simulink model "MCU_Sensing"  (R2024a)
settings: Solver=FixedStepDiscrete  StartTime=0.0  StopTime=0.0001  FixedStep=1e-7  RelTol=1e-3
libraries: fl_lib x11, slpidlib x3, simulink x3, nesl_utility x3, spsPWMGeneratorDCDCLib x1, ee_lib x1
settings Model: Creator=g_lautur  LastModifiedBy=g_lautur

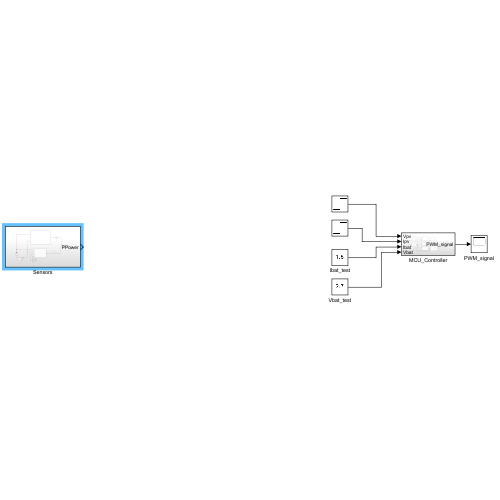
[thumbnail: Simulink's stored preview of the top-level diagram]
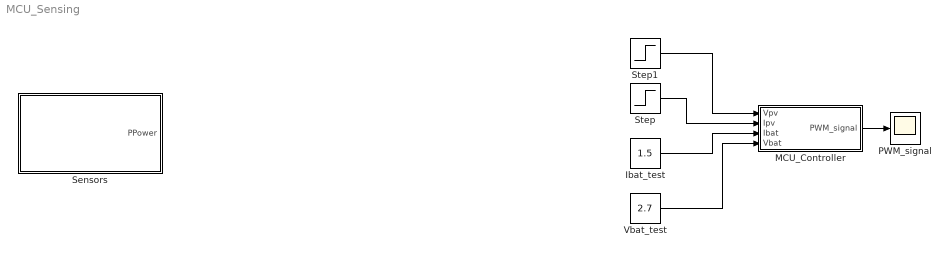
== system MCU_Sensing ==
  Ibat_test : Constant  Value=1.5
  MCU_Controller : Subsystem
  PWM_signal : Scope
  Sensors : Subsystem
  Step : Step  Time=2  Before=1.248  After=1.30  SampleTime=0
  Step1 : Step  Time=2  Before=2.0625  After=2.125  SampleTime=0
  Vbat_test : Constant  Value=2.7
  wires:
  Step1/1 -> MCU_Controller/1(Vpv)
  Step/1 -> MCU_Controller/2(Ipv)
  Vbat_test/1 -> MCU_Controller/4(Vbat)
  Ibat_test/1 -> MCU_Controller/3(Ibat)
  MCU_Controller/1(PWM_signal) -> PWM_signal/1

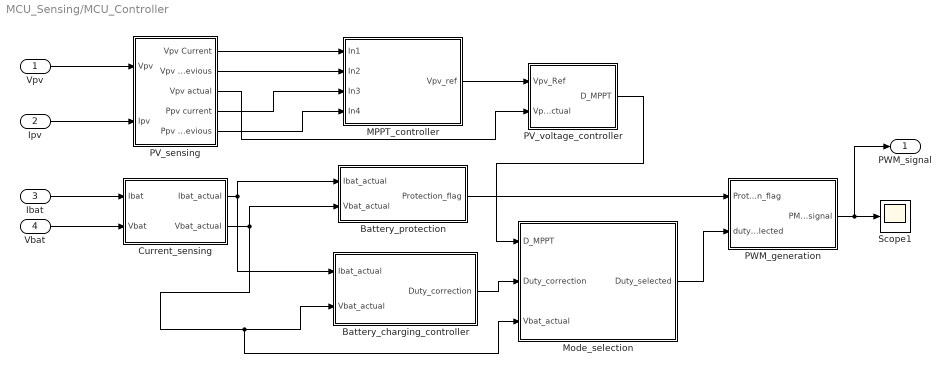
== system MCU_Sensing/MCU_Controller ==
  Vpv : Inport
  Ipv : Inport  Port=2
  Ibat : Inport  Port=3
  Vbat : Inport  Port=4
  Battery_charging_controller : Subsystem
  Battery_protection : Subsystem
  Current_sensing : Subsystem
  MPPT_controller : Subsystem
  Mode_selection : Subsystem
  PV_sensing : Subsystem
  PV_voltage_controller : Subsystem
  PWM_generation : Subsystem
  Scope1 : Scope
  PWM_signal : Outport
  wires:
  Vpv/1 -> PV_sensing/1(Vpv)
  Ipv/1 -> PV_sensing/2(Ipv)
  PV_sensing/1(Vpv Current) -> MPPT_controller/1(In1)
  PV_sensing/2(Vpv Previous) -> MPPT_controller/2(In2)
  PV_sensing/4(Ppv current) -> MPPT_controller/3(In3)
  PV_sensing/5(Ppv previous) -> MPPT_controller/4(In4)
  MPPT_controller/1(Vpv_ref) -> PV_voltage_controller/1(Vpv_Ref)
  PV_sensing/3(Vpv actual) -> PV_voltage_controller/2(Vpv_actual)
  Current_sensing/1(Ibat_actual) -> Battery_charging_controller/1(Ibat_actual), Battery_protection/1(Ibat_actual)
  Current_sensing/2(Vbat_actual) -> Battery_charging_controller/2(Vbat_actual), Mode_selection/3(Vbat_actual), Battery_protection/2(Vbat_actual)
  Ibat/1 -> Current_sensing/1(Ibat)
  Vbat/1 -> Current_sensing/2(Vbat)
  PV_voltage_controller/1(D_MPPT) -> Mode_selection/1(D_MPPT)
  Battery_charging_controller/1(Duty_correction) -> Mode_selection/2(Duty_correction)
  Battery_protection/1(Protection_flag) -> PWM_generation/1(Protection_flag)
  Mode_selection/1(Duty_selected) -> PWM_generation/2(duty_selected)
  PWM_generation/1(PMW_signal) -> PWM_signal/1, Scope1/1

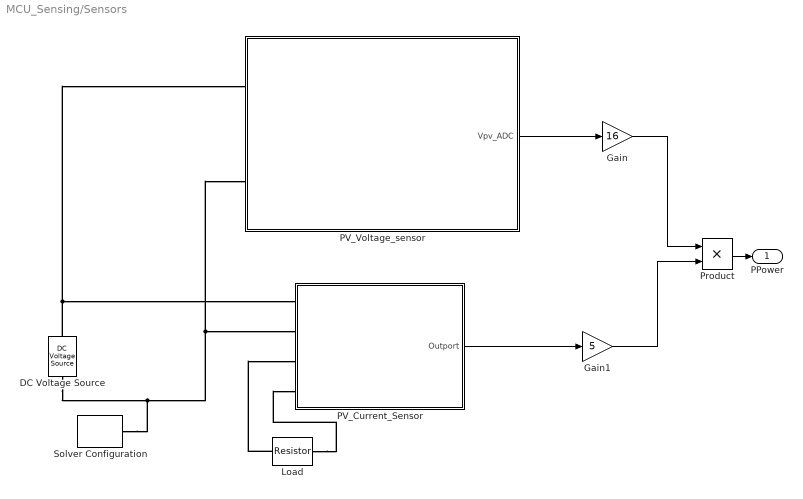
== system MCU_Sensing/Sensors ==
  DC Voltage Source : ee_lib/Additional Components/SPICE Sources/DC Voltage Source  DC=33 V
  Gain : Gain  Gain=16
  Gain1 : Gain  Gain=5
  Load : fl_lib/Electrical/Electrical Elements/Resistor  R=3.3 Ohm  i_specify=off  i_priority=None  i=0 A  i_nominal_specify=off  i_nominal_value=1  i_nominal_unit=A  v_specify=off  v_priority=None  v=0 V  v_nominal_specify=off  v_nominal_value=1  v_nominal_unit=V
  PV_Current_Sensor : Subsystem
  PV_Voltage_sensor : Subsystem
  Product : Product
  Solver Configuration : nesl_utility/Solver Configuration  PhysicalDomain=network_engine_domain  SubClassName=solver  LeftPortType=input  RightPortType=generic  Tones=[]  Harmonics=[]  SimulateNoise=off  Profile=off  UseLocalSampling=off  EnableSwitchedLinearOptims=on  FrequencyDomain=off  UseCCode=off  RelTol=0.001  AbsTol=0.001  MinStep=1e-09  ToWorkspace=off  RevertToSquareIcSolve=off  NumHomotopyIterations=100  PhasorMode=off  PhasorModeNumHarmonics=1  ConsistencySolver=NEWTON_XTOL_AFTER_FTOL  IndexReductionMethod=DerivativeReplacement  DoDC=off  ResidualTolerance=1e-09  ConsistencyTolSource=GLOBAL  ConsistencyAbsTol=0.001  ConsistencyRelTol=0.001  ConsistencyTolFactor=0.001  UseLocalSolver=off  LocalSolverChoice=NE_BACKWARD_EULER_ADVANCER  ResolveIndetEquations=on  FunctionEvalNumThread=1  LocalSolverSampleTime=0.001  DoFixedCost=off  MaxNonlinIter=3  MaxModeIter=2  ComputeImpulses=off  ImpulseIterations=2  LinearAlgebra=auto  LinearAlgebraNumThread=0  EquationFormulation=NE_TIME_EF  DelaysMemoryBudget=1024  AutomaticFiltering=on  FilteringTimeConstant=0.001  PartitionStorageMethod=AS_NEEDED  PartitionMemoryBudget=1024  PartitionMethod=ROBUST  MultibodyUseLocalSolver=off  MultibodyLocalSolverChoice=ODE1  MultibodyLocalSolverSampleTime=0.001
  PPower : Outport
  wires:
  PV_Current_Sensor/1(Outport) -> Gain1/1
  PV_Voltage_sensor/1(Vpv_ADC) -> Gain/1
  Gain1/1 -> Product/2
  Gain/1 -> Product/1
  Product/1 -> PPower/1
  connections:
  Load/RConn1 -- PV_Current_Sensor/LConn4
  DC Voltage Source/LConn1 -- PV_Current_Sensor/LConn1 -- PV_Voltage_sensor/LConn1
  Load/LConn1 -- PV_Current_Sensor/LConn3
  DC Voltage Source/RConn1 -- Solver Configuration/RConn1 -- PV_Current_Sensor/LConn2 -- PV_Voltage_sensor/LConn2

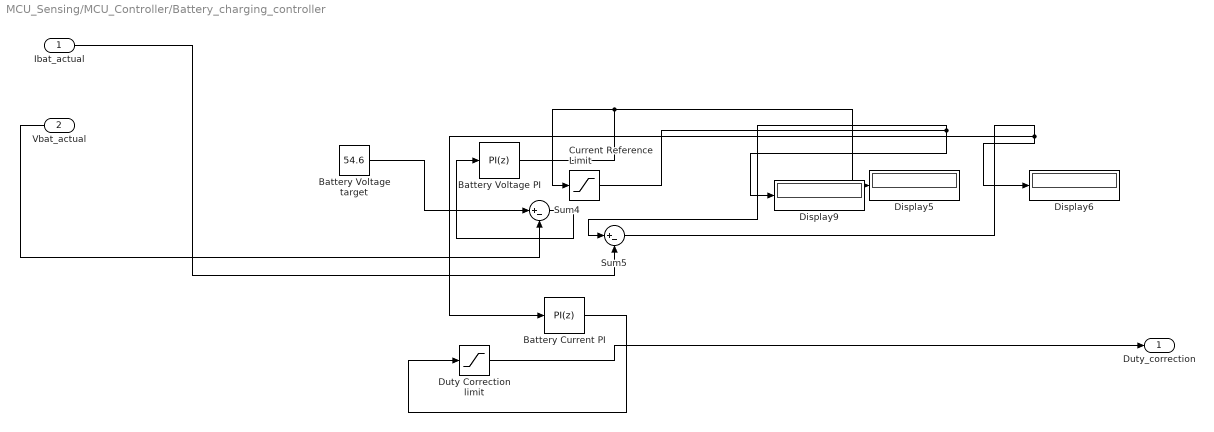
== system MCU_Sensing/MCU_Controller/Battery_charging_controller ==
  Ibat_actual : Inport
  Vbat_actual : Inport  Port=2
  "Battery Current PI " : slpidlib/PID Controller  Controller=PI  Form=Parallel  TimeDomain=Discrete-time  UseExternalTs=off  SampleTime=1e-5  IntegratorMethod=Forward Euler  FilterMethod=Forward Euler  ControllerParametersSource=internal  P=0.01  I=0.1  UseKiTs=off  D=0  UseExternalDerivativeSource=off  N=100  UseFilter=on  TunerSelectOption=Transfer Function Based (PID Tuner App)  InitialConditionSource=internal  InitialConditionForIntegrator=0  InitialConditionForFilter=0  DifferentiatorICPrevScaledInput=0  ExternalReset=none  TrackingMode=off  Kt=1  LimitOutput=off  SatLimitsSource=internal  UpperSaturationLimit=inf  LowerSaturationLimit=-inf  LinearizeAsGain=off  AntiWindupMode=none  Kb=1  LimitIntegrator=off  UpperIntegratorSaturationLimit=inf  LowerIntegratorSaturationLimit=-inf  POutMin=[]  POutMax=[]  IOutMin=[]  IOutMax=[]  DOutMin=[]  DOutMax=[]  NOutMin=[]  NOutMax=[]  SumOutMin=[]  SumOutMax=[]  SaturationOutMin=[]  SaturationOutMax=[]  PParamMin=[]  PParamMax=[]  IParamMin=[]  IParamMax=[]  DParamMin=[]  DParamMax=[]  NParamMin=[]  NParamMax=[]  KbParamMin=[]  KbParamMax=[]  KtParamMin=[]  KtParamMax=[]  KbOutMin=[]  KbOutMax=[]  KtOutMin=[]  KtOutMax=[]  IntegratorOutMin=[]  IntegratorOutMax=[]  FilterOutMin=[]  FilterOutMax=[]  SumI1OutMin=[]  SumI1OutMax=[]  SumI2OutMin=[]  SumI2OutMax=[]  SumI3OutMin=[]  SumI3OutMax=[]  SumI4OutMin=[]  SumI4OutMax=[]  SumDOutMin=[]  SumDOutMax=[]  DifferentiatorOutMin=[]  DifferentiatorOutMax=[]  FilterDiffOutCoefMin=[]  FilterDiffOutCoefMax=[]  ReciprocalOutMin=[]  ReciprocalOutMax=[]  SumDenOutMin=[]  SumDenOutMax=[]  SumNumOutMin=[]  SumNumOutMax=[]  DivideOutMin=[]  DivideOutMax=[]  UdiffTsProdOutMin=[]  UdiffTsProdOutMax=[]  NTsProdOutMin=[]  NTsProdOutMax=[]  UintegralTsProdOutMin=[]  UintegralTsProdOutMax=[]  UngainTsProdOutMin=[]  UngainTsProdOutMax=[]  ClampingZeroOutDataTypeStr=Inherit: Inherit via back propagation  ClampingZeroOutMin=[]  ClampingZeroOutMax=[]  FilterDenConstantOutDataTypeStr=Inherit: Inherit via back propagation  FilterDenConstantOutMin=[]  FilterDenConstantOutMax=[]  PCopyOutDataTypeStr=Inherit: Inherit via back propagation  PCopyOutMin=[]  PCopyOutMax=[]  NCopyOutDataTypeStr=Inherit: Inherit via back propagation  NCopyOutMin=[]  NCopyOutMax=[]  IntegratorContinuousStateAttributes=''  IntegratorStateMustResolveToSignalObject=off  IntegratorRTWStateStorageClass=Auto  FilterContinuousStateAttributes=''  FilterStateMustResolveToSignalObject=off  FilterRTWStateStorageClass=Auto  ParallelPVariant=InternalParameters  IdealPVariant=Disabled  IVariant=InternalParameters  DVariant=Disabled  IntegratorVariant=Discrete  SatVariant=Disabled  AWVariant=Passthrough  PCopyVariant=Disabled  TRVariant=Disabled  FdbkBlocksVariant=Forward  IdealPFdbkVariant=Disabled  SatFdbkVariant=Disabled  DerivativeFilterVariant=Disabled  NVariant=Disabled  NCopyVariant=Disabled_SignalSpec  FilterICVariant=Disabled  IntegratorICVariant=InternalICs  ExternalResetVariant=Disabled  TRSumVariant=Passthrough  SumFdbkVariant=Disabled  SumVariant=Sum_PI  TsampFilterVariant=InternalTs  TsampNgainVariant=Passthrough  TsampIntegralVariant=Disabled_SignalSpec  ExternalSaturationOutDataTypeStr=Inherit: Same as second input  DerivativeSourceVariant=Disabled
      settings: LibrarySourceBlock=simulink/Discrete/Discrete PID Controller
  Battery Voltage PI : slpidlib/PID Controller  Controller=PI  Form=Parallel  TimeDomain=Discrete-time  UseExternalTs=off  SampleTime=1e-5  IntegratorMethod=Forward Euler  FilterMethod=Forward Euler  ControllerParametersSource=internal  P=2  I=0.1  UseKiTs=off  D=0  UseExternalDerivativeSource=off  N=100  UseFilter=on  TunerSelectOption=Transfer Function Based (PID Tuner App)  InitialConditionSource=internal  InitialConditionForIntegrator=0  InitialConditionForFilter=0  DifferentiatorICPrevScaledInput=0  ExternalReset=none  TrackingMode=off  Kt=1  LimitOutput=off  SatLimitsSource=internal  UpperSaturationLimit=inf  LowerSaturationLimit=-inf  LinearizeAsGain=off  AntiWindupMode=none  Kb=1  LimitIntegrator=off  UpperIntegratorSaturationLimit=inf  LowerIntegratorSaturationLimit=-inf  POutMin=[]  POutMax=[]  IOutMin=[]  IOutMax=[]  DOutMin=[]  DOutMax=[]  NOutMin=[]  NOutMax=[]  SumOutMin=[]  SumOutMax=[]  SaturationOutMin=[]  SaturationOutMax=[]  PParamMin=[]  PParamMax=[]  IParamMin=[]  IParamMax=[]  DParamMin=[]  DParamMax=[]  NParamMin=[]  NParamMax=[]  KbParamMin=[]  KbParamMax=[]  KtParamMin=[]  KtParamMax=[]  KbOutMin=[]  KbOutMax=[]  KtOutMin=[]  KtOutMax=[]  IntegratorOutMin=[]  IntegratorOutMax=[]  FilterOutMin=[]  FilterOutMax=[]  SumI1OutMin=[]  SumI1OutMax=[]  SumI2OutMin=[]  SumI2OutMax=[]  SumI3OutMin=[]  SumI3OutMax=[]  SumI4OutMin=[]  SumI4OutMax=[]  SumDOutMin=[]  SumDOutMax=[]  DifferentiatorOutMin=[]  DifferentiatorOutMax=[]  FilterDiffOutCoefMin=[]  FilterDiffOutCoefMax=[]  ReciprocalOutMin=[]  ReciprocalOutMax=[]  SumDenOutMin=[]  SumDenOutMax=[]  SumNumOutMin=[]  SumNumOutMax=[]  DivideOutMin=[]  DivideOutMax=[]  UdiffTsProdOutMin=[]  UdiffTsProdOutMax=[]  NTsProdOutMin=[]  NTsProdOutMax=[]  UintegralTsProdOutMin=[]  UintegralTsProdOutMax=[]  UngainTsProdOutMin=[]  UngainTsProdOutMax=[]  ClampingZeroOutDataTypeStr=Inherit: Inherit via back propagation  ClampingZeroOutMin=[]  ClampingZeroOutMax=[]  FilterDenConstantOutDataTypeStr=Inherit: Inherit via back propagation  FilterDenConstantOutMin=[]  FilterDenConstantOutMax=[]  PCopyOutDataTypeStr=Inherit: Inherit via back propagation  PCopyOutMin=[]  PCopyOutMax=[]  NCopyOutDataTypeStr=Inherit: Inherit via back propagation  NCopyOutMin=[]  NCopyOutMax=[]  IntegratorContinuousStateAttributes=''  IntegratorStateMustResolveToSignalObject=off  IntegratorRTWStateStorageClass=Auto  FilterContinuousStateAttributes=''  FilterStateMustResolveToSignalObject=off  FilterRTWStateStorageClass=Auto  ParallelPVariant=InternalParameters  IdealPVariant=Disabled  IVariant=InternalParameters  DVariant=Disabled  IntegratorVariant=Discrete  SatVariant=Disabled  AWVariant=Passthrough  PCopyVariant=Disabled  TRVariant=Disabled  FdbkBlocksVariant=Forward  IdealPFdbkVariant=Disabled  SatFdbkVariant=Disabled  DerivativeFilterVariant=Disabled  NVariant=Disabled  NCopyVariant=Disabled_SignalSpec  FilterICVariant=Disabled  IntegratorICVariant=InternalICs  ExternalResetVariant=Disabled  TRSumVariant=Passthrough  SumFdbkVariant=Disabled  SumVariant=Sum_PI  TsampFilterVariant=InternalTs  TsampNgainVariant=Passthrough  TsampIntegralVariant=Disabled_SignalSpec  ExternalSaturationOutDataTypeStr=Inherit: Same as second input  DerivativeSourceVariant=Disabled
      settings: LibrarySourceBlock=simulink/Discrete/Discrete PID Controller
  Battery Voltage target : Constant  Value=54.6
  Current Reference Limit : Saturate  UpperLimit=8  LowerLimit=0
  Display5 : Display
  Display6 : Display
  Display9 : Display
  Duty Correction limit : Saturate  UpperLimit=0.8  LowerLimit=-0.8
  Sum4 : Sum  Inputs=|+-
  Sum5 : Sum  Inputs=|+-
  Duty_correction : Outport
  wires:
  Sum4/1 -> Battery Voltage PI/1
  Battery Voltage PI/1 -> Display5/1, Current Reference Limit/1
  Duty Correction limit/1 -> Duty_correction/1
  Battery Voltage target/1 -> Sum4/1
  Current Reference Limit/1 -> Sum5/1, Display9/1
  Sum5/1 -> "Battery Current PI "/1, Display6/1
  "Battery Current PI "/1 -> Duty Correction limit/1
  Ibat_actual/1 -> Sum5/2
  Vbat_actual/1 -> Sum4/2

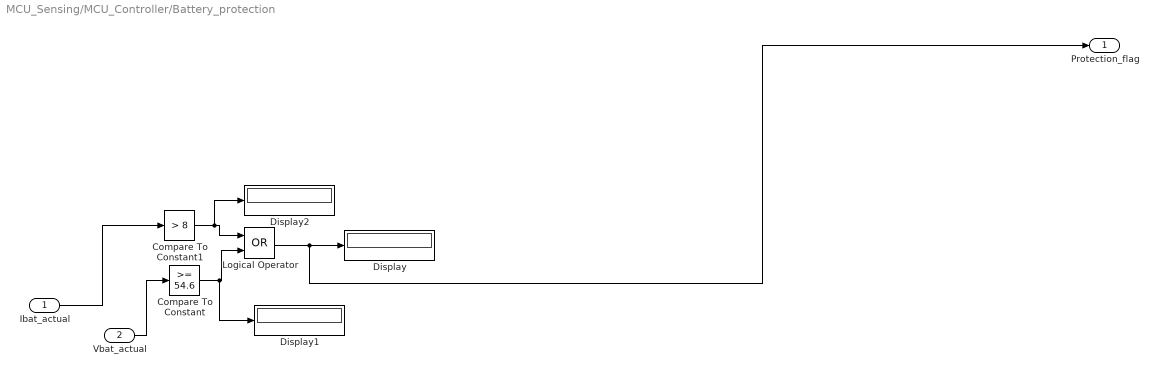
== system MCU_Sensing/MCU_Controller/Battery_protection ==
  Ibat_actual : Inport
  Vbat_actual : Inport  Port=2
  Compare To Constant : simulink/Logic and Bit Operations/Compare To Constant  relop=>=  const=54.6  OutDataTypeStr=boolean
  Compare To Constant1 : simulink/Logic and Bit Operations/Compare To Constant  relop=>  const=8  OutDataTypeStr=boolean  ZeroCross=off
  Display : Display
  Display1 : Display
  Display2 : Display
  Logical Operator : Logic  Operator=OR  AllPortsSameDT=off  OutDataTypeStr=boolean
  Protection_flag : Outport
  wires:
  Compare To Constant/1 -> Display1/1, Logical Operator/2
  Compare To Constant1/1 -> Display2/1, Logical Operator/1
  Logical Operator/1 -> Protection_flag/1, Display/1
  Vbat_actual/1 -> Compare To Constant/1
  Ibat_actual/1 -> Compare To Constant1/1

== system MCU_Sensing/MCU_Controller/Current_sensing ==
  Ibat : Inport
  Vbat : Inport  Port=2
  Gain2 : Gain  Gain=5
  Gain3 : Gain  Gain=20
  Ibat_actual : Outport
  Vbat_actual : Outport  Port=2
  wires:
  Gain3/1 -> Vbat_actual/1
  Vbat/1 -> Gain3/1
  Gain2/1 -> Ibat_actual/1
  Ibat/1 -> Gain2/1

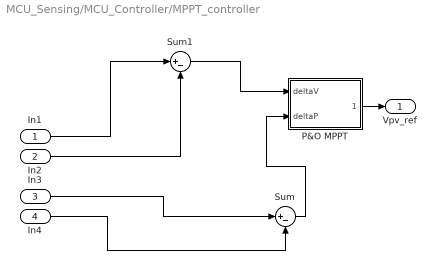
== system MCU_Sensing/MCU_Controller/MPPT_controller ==
  In1 : Inport
  In2 : Inport  Port=2
  In3 : Inport  Port=3
  In4 : Inport  Port=4
  P&O MPPT : MATLAB Function  TreatAsAtomicUnit=on
  Sum : Sum  Inputs=|+-
  Sum1 : Sum  Inputs=|+-
  Vpv_ref : Outport
  wires:
  Sum/1 -> P&O MPPT/2(deltaP)
  Sum1/1 -> P&O MPPT/1(deltaV)
  In4/1 -> Sum/2
  In1/1 -> Sum1/1
  P&O MPPT/1(Vpv_ref) -> Vpv_ref/1
  In3/1 -> Sum/1
  In2/1 -> Sum1/2

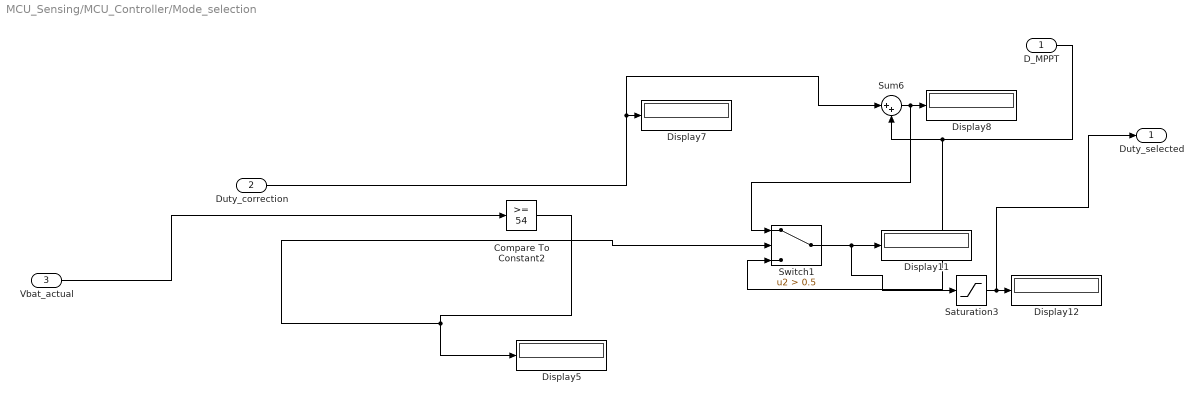
== system MCU_Sensing/MCU_Controller/Mode_selection ==
  D_MPPT : Inport
  Duty_correction : Inport  Port=2
  Vbat_actual : Inport  Port=3
  Compare To Constant2 : simulink/Logic and Bit Operations/Compare To Constant  relop=>=  const=54  OutDataTypeStr=boolean
  Display{5,7..8,11..12} (5 alike) : Display
  Saturation3 : Saturate  UpperLimit=0.8  LowerLimit=0
  Sum6 : Sum  Inputs=|++
  Switch1 : Switch  Criteria=u2 > Threshold  Threshold=0.5  SaturateOnIntegerOverflow=off  InputSameDT=off
  Duty_selected : Outport
  wires:
  D_MPPT/1 -> Switch1/3, Sum6/2
  Sum6/1 -> Switch1/1, Display8/1
  Vbat_actual/1 -> Compare To Constant2/1
  Duty_correction/1 -> Sum6/1, Display7/1
  Compare To Constant2/1 -> Display5/1, Switch1/2
  Switch1/1 -> Saturation3/1, Display11/1
  Saturation3/1 -> Duty_selected/1, Display12/1

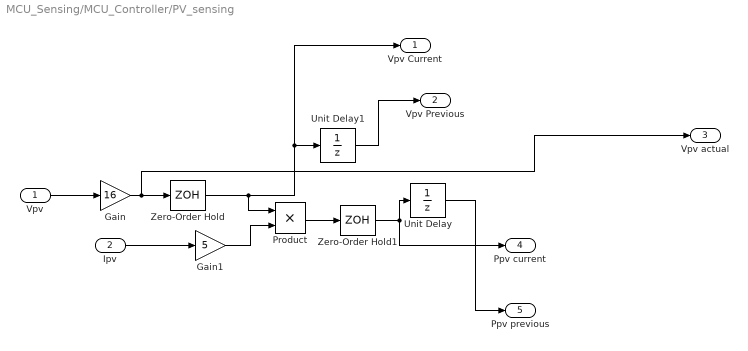
== system MCU_Sensing/MCU_Controller/PV_sensing ==
  Vpv : Inport
  Ipv : Inport  Port=2
  Gain : Gain  Gain=16
  Gain1 : Gain  Gain=5
  Product : Product
  Unit Delay : UnitDelay  InitialCondition=205.92  SampleTime=0.1  HasFrameUpgradeWarning=on
  Unit Delay1 : UnitDelay  InitialCondition=33  SampleTime=0.1  HasFrameUpgradeWarning=on
  Zero-Order Hold : ZeroOrderHold  SampleTime=0.1
  Zero-Order Hold1 : ZeroOrderHold  SampleTime=0.1
  Vpv Current : Outport
  Vpv Previous : Outport  Port=2
  Vpv actual : Outport  Port=3
  Ppv current : Outport  Port=4
  Ppv previous : Outport  Port=5
  wires:
  Product/1 -> Zero-Order Hold1/1
  Zero-Order Hold/1 -> Vpv Current/1, Unit Delay1/1, Product/1
  Unit Delay/1 -> Ppv previous/1
  Gain/1 -> Vpv actual/1, Zero-Order Hold/1
  Ipv/1 -> Gain1/1
  Gain1/1 -> Product/2
  Vpv/1 -> Gain/1
  Zero-Order Hold1/1 -> Ppv current/1, Unit Delay/1
  Unit Delay1/1 -> Vpv Previous/1

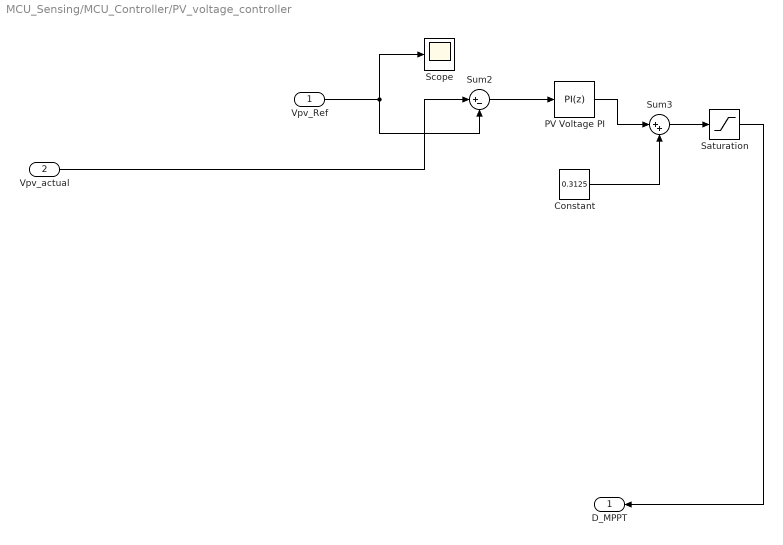
== system MCU_Sensing/MCU_Controller/PV_voltage_controller ==
  Vpv_Ref : Inport
  Vpv_actual : Inport  Port=2
  Constant : Constant  Value=0.3125
  PV Voltage PI : slpidlib/PID Controller  Controller=PI  Form=Parallel  TimeDomain=Discrete-time  UseExternalTs=off  SampleTime=0.1  IntegratorMethod=Forward Euler  FilterMethod=Forward Euler  ControllerParametersSource=internal  P=0.001  I=0.01  UseKiTs=off  D=0  UseExternalDerivativeSource=off  N=100  UseFilter=on  TunerSelectOption=Transfer Function Based (PID Tuner App)  InitialConditionSource=internal  InitialConditionForIntegrator=0  InitialConditionForFilter=0  DifferentiatorICPrevScaledInput=0  ExternalReset=none  TrackingMode=off  Kt=1  LimitOutput=off  SatLimitsSource=internal  UpperSaturationLimit=inf  LowerSaturationLimit=-inf  LinearizeAsGain=off  AntiWindupMode=none  Kb=1  LimitIntegrator=off  UpperIntegratorSaturationLimit=inf  LowerIntegratorSaturationLimit=-inf  POutMin=[]  POutMax=[]  IOutMin=[]  IOutMax=[]  DOutMin=[]  DOutMax=[]  NOutMin=[]  NOutMax=[]  SumOutMin=[]  SumOutMax=[]  SaturationOutMin=[]  SaturationOutMax=[]  PParamMin=[]  PParamMax=[]  IParamMin=[]  IParamMax=[]  DParamMin=[]  DParamMax=[]  NParamMin=[]  NParamMax=[]  KbParamMin=[]  KbParamMax=[]  KtParamMin=[]  KtParamMax=[]  KbOutMin=[]  KbOutMax=[]  KtOutMin=[]  KtOutMax=[]  IntegratorOutMin=[]  IntegratorOutMax=[]  FilterOutMin=[]  FilterOutMax=[]  SumI1OutMin=[]  SumI1OutMax=[]  SumI2OutMin=[]  SumI2OutMax=[]  SumI3OutMin=[]  SumI3OutMax=[]  SumI4OutMin=[]  SumI4OutMax=[]  SumDOutMin=[]  SumDOutMax=[]  DifferentiatorOutMin=[]  DifferentiatorOutMax=[]  FilterDiffOutCoefMin=[]  FilterDiffOutCoefMax=[]  ReciprocalOutMin=[]  ReciprocalOutMax=[]  SumDenOutMin=[]  SumDenOutMax=[]  SumNumOutMin=[]  SumNumOutMax=[]  DivideOutMin=[]  DivideOutMax=[]  UdiffTsProdOutMin=[]  UdiffTsProdOutMax=[]  NTsProdOutMin=[]  NTsProdOutMax=[]  UintegralTsProdOutMin=[]  UintegralTsProdOutMax=[]  UngainTsProdOutMin=[]  UngainTsProdOutMax=[]  ClampingZeroOutDataTypeStr=Inherit: Inherit via back propagation  ClampingZeroOutMin=[]  ClampingZeroOutMax=[]  FilterDenConstantOutDataTypeStr=Inherit: Inherit via back propagation  FilterDenConstantOutMin=[]  FilterDenConstantOutMax=[]  PCopyOutDataTypeStr=Inherit: Inherit via back propagation  PCopyOutMin=[]  PCopyOutMax=[]  NCopyOutDataTypeStr=Inherit: Inherit via back propagation  NCopyOutMin=[]  NCopyOutMax=[]  IntegratorContinuousStateAttributes=''  IntegratorStateMustResolveToSignalObject=off  IntegratorRTWStateStorageClass=Auto  FilterContinuousStateAttributes=''  FilterStateMustResolveToSignalObject=off  FilterRTWStateStorageClass=Auto  ParallelPVariant=InternalParameters  IdealPVariant=Disabled  IVariant=InternalParameters  DVariant=Disabled  IntegratorVariant=Discrete  SatVariant=Disabled  AWVariant=Passthrough  PCopyVariant=Disabled  TRVariant=Disabled  FdbkBlocksVariant=Forward  IdealPFdbkVariant=Disabled  SatFdbkVariant=Disabled  DerivativeFilterVariant=Disabled  NVariant=Disabled  NCopyVariant=Disabled_SignalSpec  FilterICVariant=Disabled  IntegratorICVariant=InternalICs  ExternalResetVariant=Disabled  TRSumVariant=Passthrough  SumFdbkVariant=Disabled  SumVariant=Sum_PI  TsampFilterVariant=InternalTs  TsampNgainVariant=Passthrough  TsampIntegralVariant=Disabled_SignalSpec  ExternalSaturationOutDataTypeStr=Inherit: Same as second input  DerivativeSourceVariant=Disabled
      settings: LibrarySourceBlock=simulink/Discrete/Discrete PID Controller
  Saturation : Saturate  UpperLimit=0.8  LowerLimit=0
  Scope : Scope
  Sum2 : Sum  Inputs=|+-
  Sum3 : Sum  Inputs=|++
  D_MPPT : Outport
  wires:
  Vpv_Ref/1 -> Sum2/2, Scope/1
  Saturation/1 -> D_MPPT/1
  PV Voltage PI/1 -> Sum3/1
  Constant/1 -> Sum3/2
  Sum3/1 -> Saturation/1
  Vpv_actual/1 -> Sum2/1
  Sum2/1 -> PV Voltage PI/1

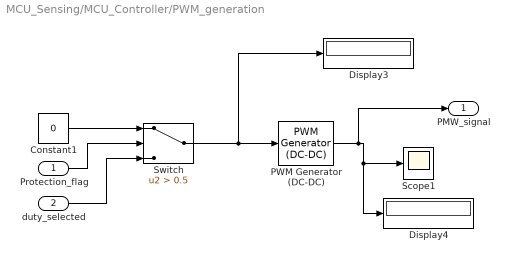
== system MCU_Sensing/MCU_Controller/PWM_generation ==
  Protection_flag : Inport
  duty_selected : Inport  Port=2
  Constant1 : Constant  Value=0
  Display3 : Display
  Display4 : Display
  PWM Generator (DC-DC) : spsPWMGeneratorDCDCLib/PWM Generator (DC-DC)  Fsw=100000  Ts=1e-7
  Scope1 : Scope
  Switch : Switch  Criteria=u2 > Threshold  Threshold=0.5  SaturateOnIntegerOverflow=off  InputSameDT=off
  PMW_signal : Outport
  wires:
  Switch/1 -> PWM Generator (DC-DC)/1, Display3/1
  duty_selected/1 -> Switch/3
  PWM Generator (DC-DC)/1 -> PMW_signal/1, Display4/1, Scope1/1
  Constant1/1 -> Switch/1
  Protection_flag/1 -> Switch/2

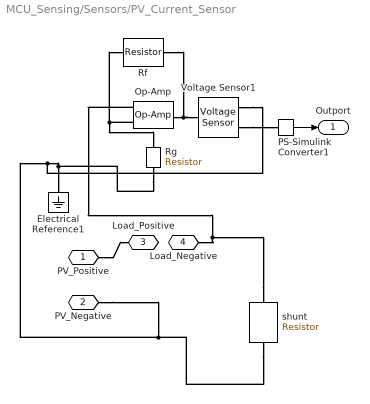
== system MCU_Sensing/Sensors/PV_Current_Sensor ==
  Electrical Reference1 : fl_lib/Electrical/Electrical Elements/Electrical Reference
  Op-Amp : fl_lib/Electrical/Electrical Elements/Op-Amp  outI_specify=off  outI_priority=None  outI=0 A  outI_nominal_specify=off  outI_nominal_value=1  outI_nominal_unit=A
  PS-Simulink Converter1 : nesl_utility/PS-Simulink Converter  PhysicalDomain=network_engine_domain  SubClassName=ps_output  LeftPortType=input  RightPortType=output  PseudoPeriodic=off  Frequencies=[]  VectorFormat=inherit  Unit=inherit  AffineConversion=off
  Rf : fl_lib/Electrical/Electrical Elements/Resistor  R=240 kOhm  i_specify=off  i_priority=None  i=0 A  i_nominal_specify=off  i_nominal_value=1  i_nominal_unit=A  v_specify=off  v_priority=None  v=0 V  v_nominal_specify=off  v_nominal_value=1  v_nominal_unit=V
  Rg : fl_lib/Electrical/Electrical Elements/Resistor  R=10 kOhm  i_specify=off  i_priority=None  i=0 A  i_nominal_specify=off  i_nominal_value=1  i_nominal_unit=A  v_specify=off  v_priority=None  v=0 V  v_nominal_specify=off  v_nominal_value=1  v_nominal_unit=V
  Voltage Sensor1 : fl_lib/Electrical/Electrical Sensors/Voltage Sensor
  shunt : fl_lib/Electrical/Electrical Elements/Resistor  R=0.005 Ohm  i_specify=off  i_priority=None  i=0 A  i_nominal_specify=off  i_nominal_value=1  i_nominal_unit=A  v_specify=off  v_priority=None  v=0 V  v_nominal_specify=off  v_nominal_value=1  v_nominal_unit=V
  PV_Positive : PMIOPort  Side=Left
  PV_Negative : PMIOPort  Port=2  Side=Left
  Load_Positive : PMIOPort  Port=3  Side=Left
  Load_Negative : PMIOPort  Port=4  Side=Left
  Outport : Outport
  wires:
  PS-Simulink Converter1/1 -> Outport/1
  connections:
  Op-Amp/RConn1 -- Rf/RConn1 -- Voltage Sensor1/LConn1
  PV_Negative/RConn1 -- shunt/RConn1 -- Voltage Sensor1/RConn2 -- Rg/RConn1 -- Electrical Reference1/LConn1
  Op-Amp/LConn2 -- Rf/LConn1 -- Rg/LConn1
  Voltage Sensor1/RConn1 -- PS-Simulink Converter1/LConn1
  shunt/LConn1 -- Load_Negative/RConn1 -- Op-Amp/LConn1
  PV_Positive/RConn1 -- Load_Positive/RConn1

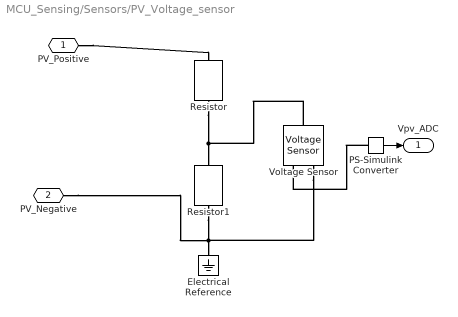
== system MCU_Sensing/Sensors/PV_Voltage_sensor ==
  Electrical Reference : fl_lib/Electrical/Electrical Elements/Electrical Reference
  PS-Simulink Converter : nesl_utility/PS-Simulink Converter  PhysicalDomain=network_engine_domain  SubClassName=ps_output  LeftPortType=input  RightPortType=output  PseudoPeriodic=off  Frequencies=[]  VectorFormat=inherit  Unit=inherit  AffineConversion=off
  Resistor : fl_lib/Electrical/Electrical Elements/Resistor  R=150 kOhm  i_specify=off  i_priority=None  i=0 A  i_nominal_specify=off  i_nominal_value=1  i_nominal_unit=A  v_specify=off  v_priority=None  v=0 V  v_nominal_specify=off  v_nominal_value=1  v_nominal_unit=V
  Resistor1 : fl_lib/Electrical/Electrical Elements/Resistor  R=10 kOhm  i_specify=off  i_priority=None  i=0 A  i_nominal_specify=off  i_nominal_value=1  i_nominal_unit=A  v_specify=off  v_priority=None  v=0 V  v_nominal_specify=off  v_nominal_value=1  v_nominal_unit=V
  Voltage Sensor : fl_lib/Electrical/Electrical Sensors/Voltage Sensor
  PV_Positive : PMIOPort  Side=Left
  PV_Negative : PMIOPort  Port=2  Side=Left
  Vpv_ADC : Outport
  wires:
  PS-Simulink Converter/1 -> Vpv_ADC/1
  connections:
  PS-Simulink Converter/LConn1 -- Voltage Sensor/RConn1
  Resistor1/RConn1 -- PV_Negative/RConn1 -- Voltage Sensor/RConn2 -- Electrical Reference/LConn1
  Resistor/RConn1 -- Voltage Sensor/LConn1 -- Resistor1/LConn1
  PV_Positive/RConn1 -- Resistor/LConn1

== matlab function MCU_Sensing/MCU_Controller/MPPT_controller/P&O MPPT ==
  data: deltaV input; Vpv_ref output; deltaP input
function Vpv_ref = fcn(deltaV, deltaP)
%#codegen

persistent voltageRef

if isempty(voltageRef)
    voltageRef = 33;  % Initial target voltage
end

step = 0.1;  % Voltage adjustment in volts

if deltaP > 0
    if deltaV > 0
        voltageRef = voltageRef + step;
    elseif deltaV < 0
        voltageRef = voltageRef - step;
    end

elseif deltaP < 0
    if deltaV > 0
        voltageRef = voltageRef - step;
    elseif deltaV < 0
        voltageRef = voltageRef + step;
    end
end

% Limit target voltage (preliminary test range)
voltageRef = min(max(voltageRef, 20), 38);

Vpv_ref = voltageRef;
